simulink model "ElectricVehicleThermalManagementWithHeatPump_2026a_version"  (R2026a)
settings: Solver=VariableStepAuto  StopTime=3600  AbsTol=1e-3
PreLoadFcn:
  | init_nmpc
InitFcn:
  | init_nmpc
model workspace: external: MATLAB File ElectricVehicleThermalManagementWithHeatPumpParameters.m (data not in the file)
values from neighbouring files (symbols this model uses):
  battery_C1_LUT = [1913.6 12447 30609 ... (first row only)    [ElectricVehicleThermalManagementWithHeatPumpParameters.m]
  battery_capacity_LUT = [280.081 276.25 276.392]    [ElectricVehicleThermalManagementWithHeatPumpParameters.m]
  battery_cell_cp = 795    [ElectricVehicleThermalManagementWithHeatPumpParameters.m]
  battery_cell_mass = 2.5    [ElectricVehicleThermalManagementWithHeatPumpParameters.m]
  battery_Em_LUT = [3.4966 3.5057 3.5148 ... (first row only)    [ElectricVehicleThermalManagementWithHeatPumpParameters.m]
  battery_N_cells = 20    [ElectricVehicleThermalManagementWithHeatPumpParameters.m]
  battery_Qe_init = 0    [ElectricVehicleThermalManagementWithHeatPumpParameters.m]
  battery_R0_LUT = [0.0117 0.0085 0.009 ... (first row only)    [ElectricVehicleThermalManagementWithHeatPumpParameters.m]
  battery_R1_LUT = [0.0109 0.0029 0.0013 ... (first row only)    [ElectricVehicleThermalManagementWithHeatPumpParameters.m]
  battery_SOC_LUT = [0; 0.1; 0.25; 0.5; 0.75; 0.9; 1]    [ElectricVehicleThermalManagementWithHeatPumpParameters.m]
  battery_T_init = -5    [ElectricVehicleThermalManagementWithHeatPumpParameters.m]
  battery_temperature_LUT = [5 20 40]    [ElectricVehicleThermalManagementWithHeatPumpParameters.m]
  cabin_duct_area = 0.04    [ElectricVehicleThermalManagementWithHeatPumpParameters.m]
  cabin_T_init = -5    [ElectricVehicleThermalManagementWithHeatPumpParameters.m]
  chiller_area_primary = 0.43982297150257105    (= 0.439822971503)    [ElectricVehicleThermalManagementWithHeatPumpParameters.m]
  chiller_N_baffles = 3    [ElectricVehicleThermalManagementWithHeatPumpParameters.m]
  chiller_N_tubes = 100    [ElectricVehicleThermalManagementWithHeatPumpParameters.m]
  chiller_tube_D = 0.0035    [ElectricVehicleThermalManagementWithHeatPumpParameters.m]
  chiller_tube_L = 0.4    [ElectricVehicleThermalManagementWithHeatPumpParameters.m]
  chiller_wall_conductivity = 240    [ElectricVehicleThermalManagementWithHeatPumpParameters.m]
  chiller_wall_thickness = 0.0001    [ElectricVehicleThermalManagementWithHeatPumpParameters.m]
  cond_evap_air_area_flow = 0.3906    [ElectricVehicleThermalManagementWithHeatPumpParameters.m]
  cond_evap_air_area_primary = 1.4834999999999998    (= 1.4835)    [ElectricVehicleThermalManagementWithHeatPumpParameters.m]
  cond_evap_W = 0.015    [ElectricVehicleThermalManagementWithHeatPumpParameters.m]
  cond_evap_wall_conductivity = 240    [ElectricVehicleThermalManagementWithHeatPumpParameters.m]
  cond_evap_wall_thickness = 0.0001    [ElectricVehicleThermalManagementWithHeatPumpParameters.m]
  coolant_channel_D = 0.0092    [ElectricVehicleThermalManagementWithHeatPumpParameters.m]
  coolant_pipe_D = 0.019    [ElectricVehicleThermalManagementWithHeatPumpParameters.m]
  coolant_T_init = -5    [ElectricVehicleThermalManagementWithHeatPumpParameters.m]
  coolant_tank_area = 0.0121    [ElectricVehicleThermalManagementWithHeatPumpParameters.m]
  coolant_tank_volume = 1.25    [ElectricVehicleThermalManagementWithHeatPumpParameters.m]
  coolant_valve_D_ratio_max = 0.95    [ElectricVehicleThermalManagementWithHeatPumpParameters.m]
  coolant_valve_D_ratio_min = 0.001    [ElectricVehicleThermalManagementWithHeatPumpParameters.m]
  coolant_valve_displacement = 0.0063    [ElectricVehicleThermalManagementWithHeatPumpParameters.m]
  coolant_valve_S_max = 0.0053    [ElectricVehicleThermalManagementWithHeatPumpParameters.m]
  evaporator_air_area_flow = 0.12    [ElectricVehicleThermalManagementWithHeatPumpParameters.m]
  evaporator_air_area_primary = 0.4323    [ElectricVehicleThermalManagementWithHeatPumpParameters.m]
  evaporator_W = 0.015    [ElectricVehicleThermalManagementWithHeatPumpParameters.m]
  evaporator_wall_conductivity = 240    [ElectricVehicleThermalManagementWithHeatPumpParameters.m]
  evaporator_wall_thickness = 0.0001    [ElectricVehicleThermalManagementWithHeatPumpParameters.m]
  expansion_valve_D_ratio_max = 0.9    [ElectricVehicleThermalManagementWithHeatPumpParameters.m]
  hex_area_primary = 0.070371675440411369    (= 0.0703716754404)    [ElectricVehicleThermalManagementWithHeatPumpParameters.m]
  hex_N_tubes = 64    [ElectricVehicleThermalManagementWithHeatPumpParameters.m]
  hex_tube_D = 0.0035    [ElectricVehicleThermalManagementWithHeatPumpParameters.m]
  hex_wall_conductivity = 240    [ElectricVehicleThermalManagementWithHeatPumpParameters.m]
  hex_wall_thickness = 0.0001    [ElectricVehicleThermalManagementWithHeatPumpParameters.m]
  inner_cond_air_area_flow = 0.1953    [ElectricVehicleThermalManagementWithHeatPumpParameters.m]
  inner_cond_air_area_primary = 0.99520000000000008    (= 0.9952)    [ElectricVehicleThermalManagementWithHeatPumpParameters.m]
  inner_cond_W = 0.02    [ElectricVehicleThermalManagementWithHeatPumpParameters.m]
  inner_cond_wall_conductivity = 240    [ElectricVehicleThermalManagementWithHeatPumpParameters.m]
  inner_cond_wall_thickness = 0.0001    [ElectricVehicleThermalManagementWithHeatPumpParameters.m]
  pump_speed_max = 1000    [ElectricVehicleThermalManagementWithHeatPumpParameters.m]
  radiator_air_area_flow = 0.097499999999999989    (= 0.0975)    [ElectricVehicleThermalManagementWithHeatPumpParameters.m]
  radiator_air_area_primary = 0.43687499999999996    (= 0.436875)    [ElectricVehicleThermalManagementWithHeatPumpParameters.m]
  radiator_W = 0.015    [ElectricVehicleThermalManagementWithHeatPumpParameters.m]
  radiator_wall_conductivity = 240    [ElectricVehicleThermalManagementWithHeatPumpParameters.m]
  radiator_wall_thickness = 0.0001    [ElectricVehicleThermalManagementWithHeatPumpParameters.m]
  refrigerant_p_init = 0.25    [ElectricVehicleThermalManagementWithHeatPumpParameters.m]
  refrigerant_pipe_D = 0.01    [ElectricVehicleThermalManagementWithHeatPumpParameters.m]
  refrigerant_valve_D_ratio_max = 0.95    [ElectricVehicleThermalManagementWithHeatPumpParameters.m]
  refrigerant_valve_displacement = 0.005    [ElectricVehicleThermalManagementWithHeatPumpParameters.m]
libraries: fl_lib x227, nesl_utility x162, SimscapeFluids_lib x30, LiBatteryElements_lib x16, slpidlib x3, SignalEditorBlockLib x1
(part 6 of 13)

== system ElectricVehicleThermalManagementWithHeatPump_2026a_version/Inverter ==
  Controlled Heat Flow Rate Source : fl_lib/Thermal/Thermal Sources/Controlled Heat Flow Rate Source
  Coolant Jacket : SimscapeFluids_lib/Thermal Liquid/Pipes & Fittings/Pipe (TL)  dynamic_compressibility=simscape.enum.onoff.on  inertia=simscape.enum.onoff.off  num_segments=1  pipe_length=0.4 m  cross_section_geometry=fluids.thermal_liquid.pipes_fittings.enum.CrossSectionGeometry.Custom  pipe_diameter=0.1 m  pipe_inner_diameter=0.05 m  pipe_outer_diameter=0.1 m  pipe_width=0.1 m  pipe_height=0.1 m  pipe_major_axis=0.1 m  pipe_minor_axis=0.05 m  pipe_side=0.1 m  pipe_angle=30 deg  area=4 * pi * coolant_channel_D^2 / 4 m^2  Dh=coolant_channel_D m  annular_heat_transfer_walls=fluids.thermal_liquid.pipes_fittings.enum.AnnularPipeWalls.AnnularInner  elevation_spec=foundation.enum.constant_variable.constant  elevation_gain=0 m  gravity_spec=foundation.enum.constant_variable.constant  g=9.81 m/s^2  pressure_loss_spec=fluids.thermal_liquid.pipes_fittings.enum.PressureLossSpec.Haaland  local_pressure_loss_spec=fluids.thermal_liquid.pipes_fittings.enum.LocalLossSpec.AggregateLength  length_add=20 * coolant_channel_D * 4 m  loss_coefficient=0.1  roughness_spec=fluids.thermal_liquid.pipes_fittings.enum.RoughnessSpec.Custom  roughness=1.5e-5 m  Re_friction_TLU=[ 400 1000 1.5e+3 3e+3 4e+3 6e+3 1e+4 2e+4 4e+4 6e+4 1e+5 1e+8 ]  friction_factor_TLU=[ 0.264 0.112 0.07099999999999999 0.0417 0.0387 0.0268 0.025 0.0232 0.0226 0.022 0.0214 0.0214 ]  Re_lam=100  Re_tur=500  shape_factor=64  mdot_nominal=[ 0.1 1 ] kg/s  p_diff_nominal=[ 0.001 0.01 ] MPa  mdot_threshold=1e-6 kg/s  wall_spec=fluids.thermal_liquid.pipes_fittings.enum.wall_spec.rigid  vol_expansion_spec=fluids.thermal_liquid.pipes_fittings.enum.VolumeExpansionSpec.Diameter  area_pressure_gain=1e-6 m^2/MPa  static_pressure_TLU=[.1, 1] MPa  area_pressure_gain_TLU=[1e-05, 1.1e-05] m^2  material_behavior_spec=fluids.thermal_liquid.pipes_fittings.enum.PipeMaterialBehavior.Linear  diameter_pressure_gain=1.2e-6 m/MPa  wall_thickness=0.05 m  elastic_modulus=69 GPa  stress_TLU=[276, 310] MPa  strain_TLU=[.004, .02]  stress_assert_action=simscape.enum.assert.action.none  stress_max=400 MPa  poisson_ratio=0.33  wall_time_constant=0.01 s  environment_spec=foundation.enum.pressure_spec.atmospheric  environment_pressure=0.101325 MPa  thermal_expansion=false  alpha_L_wall=24 um/(deltaK*m)  thermal_expansion_Tref=293.15 K  heat_transfer_spec=fluids.thermal_liquid.pipes_fittings.enum.HeatTransferSpec.DittusBoelter  mdot_nominal_heat=[ 0.1 1 ] kg/s  T_in_nominal=[ 293.15 293.15 ] K  T_out_nominal=[ 300 300 ] K  p_in_nominal_heat=[ 0.101325 0.101325 ] MPa  T_wall_nominal=[ 303.15 303.15 ] K  T_wall_eff_nominal=[303.15, 303.15] K  a_coeff=0.3  b_Re_power=0.8  c_Pr_power=0.33  Nu_lam=3.66  Re_Colburn_TLU=[ 100 150 1000 ]  Colburn_factor_TLU=[ 0.019 0.013 0.002 ]  Re_Nu_TLU=[ 100 150 1000 ]  Pr_Nu_TLU=[ 1 10 ]  Nu_TLU=[ 3.72 4.21; 3.75 4.44; 4.21 7.15 ]  annular_correction=fluids.thermal_liquid.pipes_fittings.enum.AnnularPipeCorrectionFactor.Gnielinski  p0_vec=coolant_p_init MPa  T0_vec=coolant_T_init degC  mdot0=0.1 kg/s  p_nominal=0.101325 MPa  T_nominal=293.15 K
  Inverter : fl_lib/Thermal/Thermal Elements/Thermal Mass  mass_type=foundation.enum.constant_variable.constant  mass=1 kg  sp_heat=447 J/kg/K  mass_min=1e-6 kg  num_ports=foundation.enum.numPorts2.one  m_specify=off  m_priority=High  m=1 kg  m_nominal_specify=off  m_nominal_value=1  m_nominal_unit=kg  T_specify=on  T_priority=High  T=coolant_T_init degC  T_nominal_specify=off  T_nominal_value=1  T_nominal_unit=K  Q_specify=off  Q_priority=None  Q=0 W  Q_nominal_specify=off  Q_nominal_value=1  Q_nominal_unit=W
  PS-Simulink Converter : nesl_utility/PS-Simulink Converter  PhysicalDomain=network_engine_domain  SubClassName=ps_output  LeftPortType=input  RightPortType=output  PseudoPeriodic=off  Frequencies=[]  VectorFormat=inherit  Unit=degC  AffineConversion=on
  SC7 : Subsystem
  Scope : Scope
      settings: ActiveDisplayYMinimum=-15.64467  ActiveDisplayYMaximum=40.80204
  Simulink-PS Converter : nesl_utility/Simulink-PS Converter  PhysicalDomain=network_engine_domain  SubClassName=ps_input  LeftPortType=input  RightPortType=output  PseudoPeriodic=off  Frequencies=[]  NoiseDistribution=none  NoiseParameters=[]  Unit=W  AffineConversion=off  FilteringAndDerivatives=provide  SimscapeFilterOrder=1  InputFilterTimeConstant=0.001  UdotUserProvided=0
  Temperature Sensor : fl_lib/Thermal/Thermal Sensors/Temperature Sensor  temperature_measure=foundation.enum.MeasurementReference.absolute
  Thermal Reference : fl_lib/Thermal/Thermal Elements/Thermal Reference
  To Workspace : ToWorkspace  VariableName=Q_inverterMeas  SampleTime=-1
  To Workspace1 : ToWorkspace  VariableName=T_inverterMeas  SampleTime=-1
  A : PMIOPort  Side=Left
  B : PMIOPort  Port=2  Side=Right
  tag scope: T_inverter=global
  wires:
  [Q_inverter] -> To Workspace/1, Simulink-PS Converter/1
  PS-Simulink Converter/1 -> To Workspace1/1, Scope/1, [T_inverter]
  connections:
  Inverter/LConn1 -- Controlled Heat Flow Rate Source/LConn1 -- Temperature Sensor/LConn1 -- Coolant Jacket/LConn2
  SC7/LConn1 -- Coolant Jacket/RConn1
  Controlled Heat Flow Rate Source/RConn2 -- Thermal Reference/LConn1
  SC7/RConn1 -- B/RConn1
  PS-Simulink Converter/LConn1 -- Temperature Sensor/RConn1
  A/RConn1 -- Coolant Jacket/LConn1
  Simulink-PS Converter/RConn1 -- Controlled Heat Flow Rate Source/RConn1

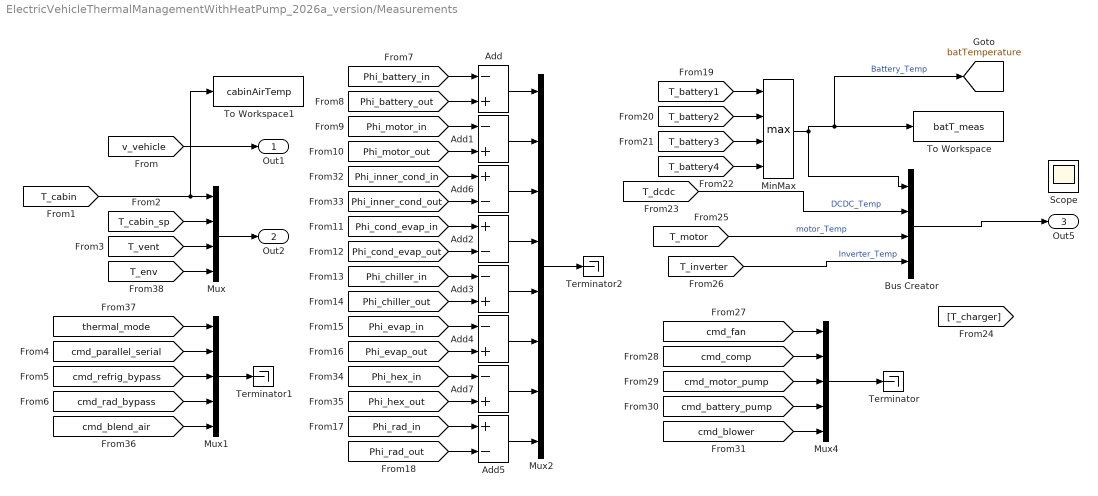
== system ElectricVehicleThermalManagementWithHeatPump_2026a_version/Measurements ==
  Add{,1,3..4,7} (5 alike) : Sum  Inputs=-+
  Add2 : Sum  Inputs=+-
  Add5 : Sum  Inputs=+-
  Add6 : Sum  Inputs=+-
  Bus Creator : BusCreator  Inputs=4
  MinMax : MinMax  Function=max  Inputs=4
  Mux : Mux
  Mux1 : Mux  Inputs=5
  Mux2 : Mux  Inputs=8
  Mux4 : Mux  Inputs=5
  Scope : Scope
      settings: ActiveDisplayYMinimum=-1  ActiveDisplayYMaximum=1  DataLoggingVariableName=ScopeData4
  Terminator : Terminator
  Terminator1 : Terminator
  Terminator2 : Terminator
  To Workspace : ToWorkspace  VariableName=batT_meas  SampleTime=-1
  To Workspace1 : ToWorkspace  VariableName=cabinAirTemp  SampleTime=-1
  Out1 : Outport
  Out2 : Outport  Port=2
  Out5 : Outport  Port=3
  tag scope: batTemperature=global
  wires:
  [v_vehicle] -> Out1/1
  [T_cabin] -> To Workspace1/1, Mux/1
  [T_cabin_sp] -> Mux/2
  [T_vent] -> Mux/3
  Mux/1 -> Out2/1
  Mux1/1 -> Terminator1/1
  [Phi_battery_in] -> Add/1
  [Phi_battery_out] -> Add/2
  [Phi_motor_in] -> Add1/1
  [Phi_motor_out] -> Add1/2
  [Phi_cond_evap_in] -> Add2/1
  [Phi_cond_evap_out] -> Add2/2
  [Phi_chiller_in] -> Add3/1
  [Phi_chiller_out] -> Add3/2
  [Phi_evap_in] -> Add4/1
  [Phi_evap_out] -> Add4/2
  [Phi_rad_in] -> Add5/1
  [Phi_rad_out] -> Add5/2
  Add/1 -> Mux2/1
  Add1/1 -> Mux2/2
  Mux2/1 -> Terminator2/1
  [T_battery1] -> MinMax/1
  [T_battery2] -> MinMax/2
  [T_battery3] -> MinMax/3
  [T_battery4] -> MinMax/4
  [T_dcdc] -> Bus Creator/2  "DCDC_Temp"
  [cmd_fan] -> Mux4/1
  [cmd_comp] -> Mux4/2
  [cmd_motor_pump] -> Mux4/3
  [cmd_battery_pump] -> Mux4/4
  [cmd_blower] -> Mux4/5
  Mux4/1 -> Terminator/1
  [Phi_inner_cond_in] -> Add6/1
  [Phi_inner_cond_out] -> Add6/2
  [Phi_hex_out] -> Add7/2
  [Phi_hex_in] -> Add7/1
  Add5/1 -> Mux2/8
  Add7/1 -> Mux2/7
  Add4/1 -> Mux2/6
  Add3/1 -> Mux2/5
  Add2/1 -> Mux2/4
  Add6/1 -> Mux2/3
  [cmd_blend_air] -> Mux1/5
  [cmd_rad_bypass] -> Mux1/4
  [cmd_refrig_bypass] -> Mux1/3
  [cmd_parallel_serial] -> Mux1/2
  [thermal_mode] -> Mux1/1
  [T_env] -> Mux/4
  MinMax/1 -> Bus Creator/1, [batTemperature], To Workspace/1  "Battery_Temp"
  [T_motor] -> Bus Creator/3  "motor_Temp"
  [T_inverter] -> Bus Creator/4  "Inverter_Temp"
  Bus Creator/1 -> Out5/1

== system ElectricVehicleThermalManagementWithHeatPump_2026a_version/Motor ==
  Controlled Heat Flow Rate Source : fl_lib/Thermal/Thermal Sources/Controlled Heat Flow Rate Source
  Coolant Jacket : SimscapeFluids_lib/Thermal Liquid/Pipes & Fittings/Pipe (TL)  dynamic_compressibility=simscape.enum.onoff.on  inertia=simscape.enum.onoff.off  num_segments=1  pipe_length=0.4 m  cross_section_geometry=fluids.thermal_liquid.pipes_fittings.enum.CrossSectionGeometry.Custom  pipe_diameter=0.1 m  pipe_inner_diameter=0.05 m  pipe_outer_diameter=0.1 m  pipe_width=0.1 m  pipe_height=0.1 m  pipe_major_axis=0.1 m  pipe_minor_axis=0.05 m  pipe_side=0.1 m  pipe_angle=30 deg  area=4 * pi * coolant_channel_D^2 / 4 m^2  Dh=coolant_channel_D m  annular_heat_transfer_walls=fluids.thermal_liquid.pipes_fittings.enum.AnnularPipeWalls.AnnularInner  elevation_spec=foundation.enum.constant_variable.constant  elevation_gain=0 m  gravity_spec=foundation.enum.constant_variable.constant  g=9.81 m/s^2  pressure_loss_spec=fluids.thermal_liquid.pipes_fittings.enum.PressureLossSpec.Haaland  local_pressure_loss_spec=fluids.thermal_liquid.pipes_fittings.enum.LocalLossSpec.AggregateLength  length_add=20 * coolant_channel_D * 4 m  loss_coefficient=0.1  roughness_spec=fluids.thermal_liquid.pipes_fittings.enum.RoughnessSpec.Custom  roughness=1.5e-5 m  Re_friction_TLU=[ 400 1000 1.5e+3 3e+3 4e+3 6e+3 1e+4 2e+4 4e+4 6e+4 1e+5 1e+8 ]  friction_factor_TLU=[ 0.264 0.112 0.07099999999999999 0.0417 0.0387 0.0268 0.025 0.0232 0.0226 0.022 0.0214 0.0214 ]  Re_lam=100  Re_tur=500  shape_factor=64  mdot_nominal=[ 0.1 1 ] kg/s  p_diff_nominal=[ 0.001 0.01 ] MPa  mdot_threshold=1e-6 kg/s  wall_spec=fluids.thermal_liquid.pipes_fittings.enum.wall_spec.rigid  vol_expansion_spec=fluids.thermal_liquid.pipes_fittings.enum.VolumeExpansionSpec.Diameter  area_pressure_gain=1e-6 m^2/MPa  static_pressure_TLU=[.1, 1] MPa  area_pressure_gain_TLU=[1e-05, 1.1e-05] m^2  material_behavior_spec=fluids.thermal_liquid.pipes_fittings.enum.PipeMaterialBehavior.Linear  diameter_pressure_gain=1.2e-6 m/MPa  wall_thickness=0.05 m  elastic_modulus=69 GPa  stress_TLU=[276, 310] MPa  strain_TLU=[.004, .02]  stress_assert_action=simscape.enum.assert.action.none  stress_max=400 MPa  poisson_ratio=0.33  wall_time_constant=0.01 s  environment_spec=foundation.enum.pressure_spec.atmospheric  environment_pressure=0.101325 MPa  thermal_expansion=false  alpha_L_wall=24 um/(deltaK*m)  thermal_expansion_Tref=293.15 K  heat_transfer_spec=fluids.thermal_liquid.pipes_fittings.enum.HeatTransferSpec.DittusBoelter  mdot_nominal_heat=[ 0.1 1 ] kg/s  T_in_nominal=[ 293.15 293.15 ] K  T_out_nominal=[ 300 300 ] K  p_in_nominal_heat=[ 0.101325 0.101325 ] MPa  T_wall_nominal=[ 303.15 303.15 ] K  T_wall_eff_nominal=[303.15, 303.15] K  a_coeff=0.3  b_Re_power=0.8  c_Pr_power=0.33  Nu_lam=3.66  Re_Colburn_TLU=[ 100 150 1000 ]  Colburn_factor_TLU=[ 0.019 0.013 0.002 ]  Re_Nu_TLU=[ 100 150 1000 ]  Pr_Nu_TLU=[ 1 10 ]  Nu_TLU=[ 3.72 4.21; 3.75 4.44; 4.21 7.15 ]  annular_correction=fluids.thermal_liquid.pipes_fittings.enum.AnnularPipeCorrectionFactor.Gnielinski  p0_vec=coolant_p_init MPa  T0_vec=coolant_T_init degC  mdot0=0.1 kg/s  p_nominal=0.101325 MPa  T_nominal=293.15 K
  Motor : fl_lib/Thermal/Thermal Elements/Thermal Mass  mass_type=foundation.enum.constant_variable.constant  mass=46 kg  sp_heat=447 J/kg/K  mass_min=1e-6 kg  num_ports=foundation.enum.numPorts2.one  m_specify=off  m_priority=High  m=1 kg  m_nominal_specify=off  m_nominal_value=1  m_nominal_unit=kg  T_specify=on  T_priority=High  T=coolant_T_init degC  T_nominal_specify=off  T_nominal_value=1  T_nominal_unit=K  Q_specify=off  Q_priority=None  Q=0 W  Q_nominal_specify=off  Q_nominal_value=1  Q_nominal_unit=W
  PS-Simulink Converter : nesl_utility/PS-Simulink Converter  PhysicalDomain=network_engine_domain  SubClassName=ps_output  LeftPortType=input  RightPortType=output  PseudoPeriodic=off  Frequencies=[]  VectorFormat=inherit  Unit=degC  AffineConversion=on
  SC5 : Subsystem
  SC6 : Subsystem
  Simulink-PS Converter : nesl_utility/Simulink-PS Converter  PhysicalDomain=network_engine_domain  SubClassName=ps_input  LeftPortType=input  RightPortType=output  PseudoPeriodic=off  Frequencies=[]  NoiseDistribution=none  NoiseParameters=[]  Unit=W  AffineConversion=off  FilteringAndDerivatives=provide  SimscapeFilterOrder=1  InputFilterTimeConstant=0.001  UdotUserProvided=0
  Temperature Sensor : fl_lib/Thermal/Thermal Sensors/Temperature Sensor  temperature_measure=foundation.enum.MeasurementReference.absolute
  Thermal Reference : fl_lib/Thermal/Thermal Elements/Thermal Reference
  To Workspace : ToWorkspace  VariableName=Q_motMeasured  SampleTime=-1
  To Workspace1 : ToWorkspace  VariableName=Motor_Temp  SampleTime=-1
  A : PMIOPort  Side=Left
  B : PMIOPort  Port=2  Side=Right
  tag scope: T_motor=global
  wires:
  PS-Simulink Converter/1 -> To Workspace1/1, [T_motor]
  [Q_motor] -> To Workspace/1, Simulink-PS Converter/1
  connections:
  Motor/LConn1 -- Coolant Jacket/LConn2 -- Controlled Heat Flow Rate Source/LConn1 -- Temperature Sensor/LConn1
  Simulink-PS Converter/RConn1 -- Controlled Heat Flow Rate Source/RConn1
  PS-Simulink Converter/LConn1 -- Temperature Sensor/RConn1
  SC6/LConn1 -- Coolant Jacket/RConn1
  SC6/RConn1 -- B/RConn1
  SC5/LConn1 -- A/RConn1
  Controlled Heat Flow Rate Source/RConn2 -- Thermal Reference/LConn1
  SC5/RConn1 -- Coolant Jacket/LConn1

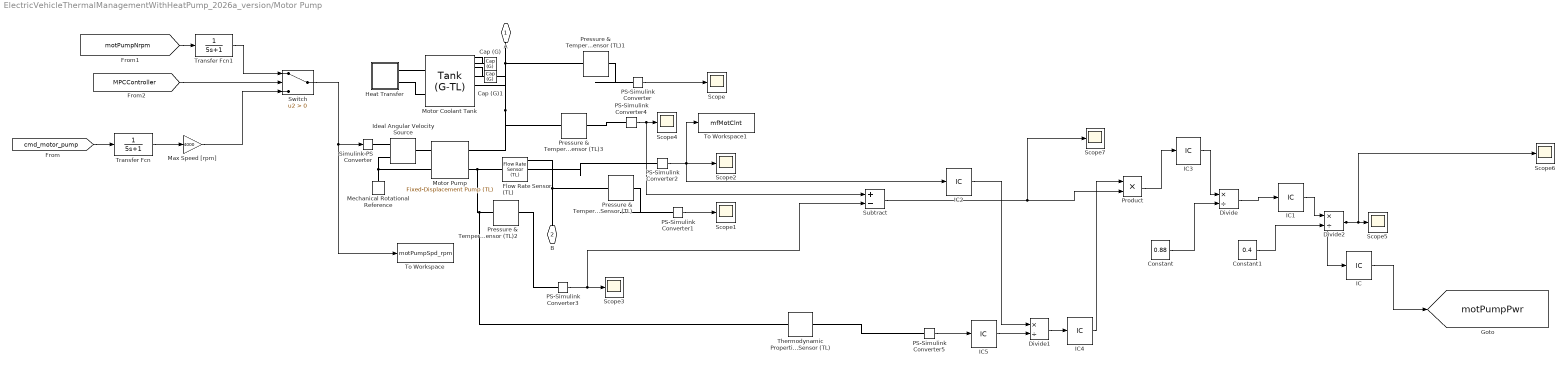
== system ElectricVehicleThermalManagementWithHeatPump_2026a_version/Motor Pump ==
  Cap (G) : fl_lib/Gas/Elements/Cap (G)  p_specify=off  p_priority=None  p=0.101325 MPa  p_nominal_specify=off  p_nominal_value=1  p_nominal_unit=MPa  T_specify=off  T_priority=None  T=293.15 K  T_nominal_specify=off  T_nominal_value=1  T_nominal_unit=K
  Cap (G)1 : fl_lib/Gas/Elements/Cap (G)  p_specify=off  p_priority=None  p=0.101325 MPa  p_nominal_specify=off  p_nominal_value=1  p_nominal_unit=MPa  T_specify=off  T_priority=None  T=293.15 K  T_nominal_specify=off  T_nominal_value=1  T_nominal_unit=K
  Constant : Constant  Value=0.88
  Constant1 : Constant  Value=0.4
  Divide : Product  Inputs=*/
  Divide1 : Product  Inputs=*/
  Divide2 : Product  Inputs=*/
  Flow Rate Sensor (TL) : fl_lib/Thermal Liquid/Sensors/Flow Rate Sensor (TL)  mass_flow_measure=true  volumetric_flow_measure=false  energy_flow_measure=true
  Heat Transfer : Subsystem
  IC{,1..4} (5 alike) : InitialCondition  Value=0
  IC5 : InitialCondition
  Ideal Angular Velocity Source : fl_lib/Mechanical/Mechanical Sources/Ideal Angular Velocity Source
  Max Speed [rpm] : Gain  Gain=4000
  Mechanical Rotational Reference : fl_lib/Mechanical/Rotational Elements/Mechanical Rotational Reference
  Motor Coolant Tank : SimscapeFluids_lib/Thermal Liquid/Tanks & Accumulators/Tank (G-TL)  num_inlet=2  volume_total=coolant_tank_volume l  volume_spec=1  tank_area=coolant_tank_area m^2  level_TLU=[0, 3, 5] m  volume_TLU=[0, 4, 6] m^3  inlet_areas_A1B1=[.01, .01] m^2  inlet_height_A2=0.1 m  inlet_area_A2=0.01 m^2  inlet_heights_A2B2=[0, 0] m  inlet_areas_A2B2=[1 1] * pi * coolant_pipe_D^2 / 4 m^2  inlet_heights_A2B2C2=[.1, .05, 0] m  inlet_areas_A2B2C2=[.01, .01, .01] m^2  inlet_heights_A2B2C2D2=0.1 * ones(1, 4) m  inlet_areas_A2B2C2D2=0.01 * ones(1, 4) m^2  inlet_heights_A2B2C2D2E2=0.1 * ones(1, 5) m  inlet_areas_A2B2C2D2E2=0.01 * ones(1, 5) m^2  inlet_heights_A2B2C2D2E2F2=0.1 * ones(1, 6) m  inlet_areas_A2B2C2D2E2F2=0.01 * ones(1, 6) m^2  capacity_check=0  max_liquid_capacity=coolant_tank_volume l  g=0 m/s^2  level_specify=on  level_priority=None  level=5 m  level_nominal_specify=off  level_nominal_value=1  level_nominal_unit=m  volume_liquid_specify=on  volume_liquid_priority=High  volume_liquid=0.25 * coolant_tank_volume l  volume_liquid_nominal_specify=off  volume_liquid_nominal_value=1  volume_liquid_nominal_unit=m^3  mass_liquid_specify=off  mass_liquid_priority=None  mass_liquid=5e+3 kg  mass_liquid_nominal_specify=off  mass_liquid_nominal_value=1  mass_liquid_nominal_unit=kg  T_liquid_specify=on  T_liquid_priority=High  T_liquid=coolant_T_init degC  T_liquid_nominal_specify=off  T_liquid_nominal_value=1  T_liquid_nominal_unit=K  p_gas_specify=on  p_gas_priority=High  p_gas=coolant_p_init MPa  p_gas_nominal_specify=off  p_gas_nominal_value=1  p_gas_nominal_unit=MPa  T_gas_specify=on  T_gas_priority=High  T_gas=coolant_T_init degC  T_gas_nominal_specify=off  T_gas_nominal_value=1  T_gas_nominal_unit=K  rho_gas_specify=off  rho_gas_priority=None  rho_gas=1.2 kg/m^3  rho_gas_nominal_specify=off  rho_gas_nominal_value=1  rho_gas_nominal_unit=kg/m^3
  Motor Pump : SimscapeFluids_lib/Thermal Liquid/Pumps & Motors/Fixed-Displacement Pump (TL)  loss_spec=1  displacement=pump_displacement l/rev  omega_nominal=0.5 * pump_speed_max rpm  p_nominal=0.1 MPa  mu_nominal=0.9 cP  vol_eff_nominal=0.92  mech_eff_nominal=0.88  no_load_torque=0.03 N*m  p_diff_eff_TLU=[.1, 1, 2] MPa  omega_eff_TLU=[25, 50, 100, 200, 300, 400] rad/s  vol_eff_TLU=[.816, .908, .954, .977, .981, .984; .325, .663, .831, .916, .925, .946; .137, .568, .78, .892, .893, .91]  mech_eff_TLU=[.996, .996, .996, .996, .996, .996; .988, .989, .989, .989, .989, .99; .981, .981, .982, .982, .983, .984]  p_diff_loss_TLU=[.1, 1, 2] MPa  omega_loss_TLU=[25, 50, 100, 200, 300, 400] rad/s  vol_loss_TLU=[.023, .023, .023, .023, .0285, .032; .0844, .0842, .0845, .084, .1125, .108; .1079, .108, .11, .108, .1605, .18] * 1e-3 m^3/s  mech_loss_TLU=[.002, .002, .002, .002, .002, .002; .0607, .0556, .0556, .0556, .0556, .0505; .1937, .1937, .1833, .1833, .1729, .1626] N*m  vol_eff_min=1e-3  vol_eff_max=1  mech_eff_min=1e-3  mech_eff_max=1  pressure_threshold=1e-3 MPa  omega_threshold=10 rad/s  area=pi * coolant_pipe_D^2 / 4 m^2  supplied_range_check=0  pump_mode_check=simscape.enum.assert.action.none  pressure_check=simscape.enum.assert.action.none  p_min_valid=0.101325 MPa
  PS-Simulink Converter{,1..5} (6 alike) : nesl_utility/PS-Simulink Converter  PhysicalDomain=network_engine_domain  SubClassName=ps_output  LeftPortType=input  RightPortType=output  PseudoPeriodic=off  Frequencies=[]  VectorFormat=inherit  Unit=inherit  AffineConversion=off
  Pressure & Temperature Sensor (TL) : fl_lib/Thermal Liquid/Sensors/Pressure & Temperature Sensor (TL)  reference=foundation.enum.MeasurementReference.absolute  pressure=false  pressure_spec=foundation.enum.PressureMeasementSpec.Absolute  temperature=true
  Pressure & Temperature Sensor (TL)1 : fl_lib/Thermal Liquid/Sensors/Pressure & Temperature Sensor (TL)  reference=foundation.enum.MeasurementReference.absolute  pressure=false  pressure_spec=foundation.enum.PressureMeasementSpec.Absolute  temperature=true
  Pressure & Temperature Sensor (TL)2 : fl_lib/Thermal Liquid/Sensors/Pressure & Temperature Sensor (TL)  reference=foundation.enum.MeasurementReference.absolute  pressure=true  pressure_spec=foundation.enum.PressureMeasementSpec.Absolute  temperature=false
  Pressure & Temperature Sensor (TL)3 : fl_lib/Thermal Liquid/Sensors/Pressure & Temperature Sensor (TL)  reference=foundation.enum.MeasurementReference.absolute  pressure=true  pressure_spec=foundation.enum.PressureMeasementSpec.Absolute  temperature=false
  Product : Product
  Scope{,1..7} (8 alike) : Scope
      Scope settings: ActiveDisplayYMinimum=263.0251  ActiveDisplayYMaximum=264.27412  DataLoggingVariableName=ScopeData3
      Scope1 settings: DataLoggingVariableName=ScopeData4
      Scope2 settings: ActiveDisplayYMinimum=-0.01351  ActiveDisplayYMaximum=0.12159  DataLoggingVariableName=ScopeData5
      Scope3 settings: ActiveDisplayYMinimum=100509.25601  ActiveDisplayYMaximum=108666.69589  DataLoggingVariableName=ScopeData3
      Scope4 settings: ActiveDisplayYMinimum=100596.97842  ActiveDisplayYMaximum=107868.3821  DataLoggingVariableName=ScopeData4
      Scope5 settings: ActiveDisplayYMinimum=-0.74504  ActiveDisplayYMaximum=0.24766  DataLoggingVariableName=ScopeData5
      Scope6 settings: DataLoggingVariableName=ScopeData7
      Scope7 settings: ActiveDisplayYMinimum=-0.74504  ActiveDisplayYMaximum=0.24766  DataLoggingVariableName=ScopeData8
  Simulink-PS Converter : nesl_utility/Simulink-PS Converter  PhysicalDomain=network_engine_domain  SubClassName=ps_input  LeftPortType=input  RightPortType=output  PseudoPeriodic=off  Frequencies=[]  NoiseDistribution=none  NoiseParameters=[]  Unit=rpm  AffineConversion=off  FilteringAndDerivatives=provide  SimscapeFilterOrder=1  InputFilterTimeConstant=0.001  UdotUserProvided=0
  Subtract : Sum  Inputs=+-
  Switch : Switch  Criteria=u2 > Threshold  SaturateOnIntegerOverflow=off  InputSameDT=off
  Thermodynamic Properties Sensor (TL) : fl_lib/Thermal Liquid/Sensors/Thermodynamic Properties Sensor (TL)  internal_energy=false  density=true  specific_heat=false
  To Workspace : ToWorkspace  VariableName=motPumpSpd_rpm  SampleTime=-1
  To Workspace1 : ToWorkspace  VariableName=mfMotClnt  SampleTime=-1
  Transfer Fcn : TransferFcn  Denominator=[5 1]
  Transfer Fcn1 : TransferFcn  Denominator=[5 1]
  A : PMIOPort  Side=Left
  B : PMIOPort  Port=2  Side=Right
  tag scope: motPumpPwr=global
  wires:
  Transfer Fcn/1 -> Max Speed [rpm]/1
  [cmd_motor_pump] -> Transfer Fcn/1
  PS-Simulink Converter/1 -> Scope/1
  PS-Simulink Converter1/1 -> Scope1/1
  PS-Simulink Converter2/1 -> IC2/1, To Workspace1/1, Scope2/1
  PS-Simulink Converter3/1 -> Subtract/2, Scope3/1
  PS-Simulink Converter4/1 -> Subtract/1, Scope4/1
  Subtract/1 -> Scope7/1, Product/2
  Product/1 -> IC3/1
  Constant/1 -> Divide/2
  Divide1/1 -> IC4/1
  Constant1/1 -> Divide2/2
  Divide2/1 -> IC/1, Scope6/1, Scope5/1
  PS-Simulink Converter5/1 -> IC5/1
  IC/1 -> [motPumpPwr]
  IC1/1 -> Divide2/1
  Divide/1 -> IC1/1
  IC2/1 -> Divide1/1
  IC3/1 -> Divide/1
  IC4/1 -> Product/1
  IC5/1 -> Divide1/2
  [motPumpNrpm] -> Transfer Fcn1/1
  [MPCController] -> Switch/2
  Max Speed [rpm]/1 -> Switch/3
  Switch/1 -> To Workspace/1, Simulink-PS Converter/1
  Transfer Fcn1/1 -> Switch/1
  connections:
  Mechanical Rotational Reference/LConn1 -- Ideal Angular Velocity Source/RConn2 -- Motor Pump/RConn2
  Ideal Angular Velocity Source/LConn1 -- Motor Pump/RConn1
  Simulink-PS Converter/RConn1 -- Ideal Angular Velocity Source/RConn1
  Pressure & Temperature Sensor (TL)/LConn1 -- Flow Rate Sensor (TL)/RConn1 -- B/RConn1
  Heat Transfer/RConn2 -- Motor Coolant Tank/RConn2
  Cap (G)/LConn1 -- Motor Coolant Tank/LConn1
  Heat Transfer/RConn1 -- Motor Coolant Tank/RConn1
  Motor Coolant Tank/LConn4 -- Pressure & Temperature Sensor (TL)3/LConn1 -- Motor Pump/LConn1
  A/RConn1 -- Pressure & Temperature Sensor (TL)1/LConn1 -- Motor Coolant Tank/LConn3
  Cap (G)1/LConn1 -- Motor Coolant Tank/LConn2
  PS-Simulink Converter/LConn1 -- Pressure & Temperature Sensor (TL)1/RConn1
  PS-Simulink Converter1/LConn1 -- Pressure & Temperature Sensor (TL)/RConn1
  Flow Rate Sensor (TL)/LConn1 -- Thermodynamic Properties Sensor (TL)/LConn1 -- Pressure & Temperature Sensor (TL)2/LConn1 -- Motor Pump/LConn2
  PS-Simulink Converter2/LConn1 -- Flow Rate Sensor (TL)/RConn2
  PS-Simulink Converter3/LConn1 -- Pressure & Temperature Sensor (TL)2/RConn1
  Pressure & Temperature Sensor (TL)3/RConn1 -- PS-Simulink Converter4/LConn1
  PS-Simulink Converter5/LConn1 -- Thermodynamic Properties Sensor (TL)/RConn1

== system ElectricVehicleThermalManagementWithHeatPump_2026a_version/Parallel-Serial Mode Valve 1 ==
  note: Parallel mode flow path: A-C
      | Serial mode flow path: A-B
  Bias : Bias  Bias=-1  SaturateOnIntegerOverflow=off
  Gain : Gain  Gain=2
  Max Valve Displacement [m] : Gain  Gain=coolant_valve_displacement
  Parallel-Serial Mode Valve : SimscapeFluids_lib/Thermal Liquid/Valves & Orifices/Directional Control Valves/3-Way Directional Valve (TL)  open_orifices_pos=fluids.thermal_liquid.valves.directional_control_valves.enum.OpenOrifices3Way.PA  open_orifices_neg=fluids.thermal_liquid.valves.directional_control_valves.enum.OpenOrifices3Way.AT  area_spec=fluids.thermal_liquid.valves.directional_control_valves.enum.area_spec.identical  valve_spec=fluids.thermal_liquid.valves.enum.orifice_spec.linear  del_S_max=coolant_valve_displacement m  area_max=pi * (coolant_valve_D_ratio_max*coolant_pipe_D)^2 / 4 m^2  del_S_TLU=[0 0.002 0.004 0.007 0.017] m  valve_area_TLU=[1e-09, 2.0352e-07, 4.0736e-05, .00011438, .00034356] m^2  del_S_flow_TLU=[0 0.002 0.004 0.007 0.017] m  p_diff_TLU=[-.1, .3, .5, .7] MPa  vol_flow_TLU=1e-3 * [1.7e-05, 2e-05, 2.6e-05; .0035, .0045, .0053; .7, .9, 1.06; 1.96, 2.5, 3; 6, 7.7, 9.13] m^3/s  mdot_TLU=[-1e-05, 1.7e-05, 2e-05, 2.6e-05; -.002, .0035, .0045, .0053; -.4, .7, .9, 1.06; -1.13, 1.96, 2.5, 3; -3.45, 6, 7.7, 9.13] kg/s  T_ref_in=293.15 K  p_ref_in=0.101325 MPa  area_leak=pi * (coolant_valve_D_ratio_min*coolant_pipe_D)^2 / 4 m^2  Cd=0.7  Re_c=150  smoothing_factor=0.01  pressure_recovery=simscape.enum.onoff.on  area=pi * coolant_pipe_D^2 / 4 m^2  S_max_PA=coolant_valve_S_max m  del_S_max_PA=coolant_valve_displacement-(coolant_valve_displacement)*(pi * (coolant_valve_D_ratio_min*coolant_pipe_D)^2 / 4)/(pi * (coolant_valve_D_ratio_max*coolant_pipe_D)^2 / 4) m  area_max_PA=pi * (coolant_valve_D_ratio_max*coolant_pipe_D)^2 / 4 m^2  del_S_TLU_PA=[0 0.002 0.004 0.007 0.017] m  valve_area_TLU_PA=[1e-09, 2.0352e-07, 4.0736e-05, .00011438, .00034356] m^2  del_S_flow_TLU_PA=[0 0.002 0.004 0.007 0.017] m  p_diff_TLU_PA=[-.1, .3, .5, .7] MPa  vol_flow_TLU_PA=1e-3 * [1.7e-05, 2e-05, 2.6e-05; .0035, .0045, .0053; .7, .9, 1.06; 1.96, 2.5, 3; 6, 7.7, 9.13] m^3/s  mdot_TLU_PA=[-1e-05, 1.7e-05, 2e-05, 2.6e-05; -.002, .0035, .0045, .0053; -.4, .7, .9, 1.06; -1.13, 1.96, 2.5, 3; -3.45, 6, 7.7, 9.13] kg/s  S_max_AT=-coolant_valve_S_max m  del_S_max_AT=coolant_valve_displacement-(coolant_valve_displacement)*(pi * (coolant_valve_D_ratio_min*coolant_pipe_D)^2 / 4)/(pi * (coolant_valve_D_ratio_max*coolant_pipe_D)^2 / 4) m  area_max_AT=pi * (coolant_valve_D_ratio_max*coolant_pipe_D)^2 / 4 m^2  del_S_TLU_AT=[0 0.002 0.004 0.007 0.017] m  valve_area_TLU_AT=[1e-09, 2.0352e-07, 4.0736e-05, .00011438, .00034356] m^2  del_S_flow_TLU_AT=[0 0.002 0.004 0.007 0.017] m  p_diff_TLU_AT=[-.1, .3, .5, .7] MPa  vol_flow_TLU_AT=1e-3 * [1.7e-05, 2e-05, 2.6e-05; .0035, .0045, .0053; .7, .9, 1.06; 1.96, 2.5, 3; 6, 7.7, 9.13] m^3/s  mdot_TLU_AT=[-1e-05, 1.7e-05, 2e-05, 2.6e-05; -.002, .0035, .0045, .0053; -.4, .7, .9, 1.06; -1.13, 1.96, 2.5, 3; -3.45, 6, 7.7, 9.13] kg/s  S_max_PT=2.5e-3 m  del_S_max_PT=0.005 m  area_max_PT=1e-4 m^2  del_S_TLU_PT=[0, .002, .004, .007, .017] m  valve_area_TLU_PT=[1e-09, 2.0352e-07, 4.0736e-05, .00011438, .00034356] m^2  del_S_flow_TLU_PT=[0, .002, .004, .007, .017] m  p_diff_TLU_PT=[.3, .5, .7] MPa  vol_flow_TLU_PT=1e-3 * [1.7e-05, 2e-05, 2.6e-05; .0035, .0045, .0053; .7, .9, 1.06; 1.96, 2.5, 3; 6, 7.7, 9.13] m^3/s  mdot_TLU_PT=[1.7e-05, 2e-05, 2.6e-05; .0035, .0045, .0053; .7, .9, 1.06; 1.96, 2.5, 3; 6, 7.7, 9.13] kg/s
  Simulink-PS Converter : nesl_utility/Simulink-PS Converter  PhysicalDomain=network_engine_domain  SubClassName=ps_input  LeftPortType=input  RightPortType=output  PseudoPeriodic=off  Frequencies=[]  NoiseDistribution=none  NoiseParameters=[]  Unit=m  AffineConversion=off  FilteringAndDerivatives=provide  SimscapeFilterOrder=1  InputFilterTimeConstant=0.001  UdotUserProvided=0
  Transfer Fcn : TransferFcn  Denominator=[1 1]
  C : PMIOPort  Side=Left
  A : PMIOPort  Port=2  Side=Right
  B : PMIOPort  Port=3  Side=Right
  wires:
  Gain/1 -> Bias/1
  Transfer Fcn/1 -> Gain/1
  [cmd_parallel_serial] -> Transfer Fcn/1
  Max Valve Displacement [m]/1 -> Simulink-PS Converter/1
  Bias/1 -> Max Valve Displacement [m]/1
  connections:
  Parallel-Serial Mode Valve/RConn1 -- Simulink-PS Converter/RConn1
  Parallel-Serial Mode Valve/RConn3 -- C/RConn1
  Parallel-Serial Mode Valve/LConn1 -- A/RConn1
  Parallel-Serial Mode Valve/RConn2 -- B/RConn1

== system ElectricVehicleThermalManagementWithHeatPump_2026a_version/Parallel-Serial Mode Valve 2 ==
  note: Parallel mode flow path: A-C
      | Serial mode flow path: A-B
  Bias : Bias  Bias=-1  SaturateOnIntegerOverflow=off
  Flow Rate Sensor (TL) : fl_lib/Thermal Liquid/Sensors/Flow Rate Sensor (TL)  mass_flow_measure=true  volumetric_flow_measure=false  energy_flow_measure=true
  Gain : Gain  Gain=2
  Max Valve Displacement [m] : Gain  Gain=coolant_valve_displacement
  PS-Simulink Converter : nesl_utility/PS-Simulink Converter  PhysicalDomain=network_engine_domain  SubClassName=ps_output  LeftPortType=input  RightPortType=output  PseudoPeriodic=off  Frequencies=[]  VectorFormat=inherit  Unit=inherit  AffineConversion=off
  Parallel-Serial Mode Valve : SimscapeFluids_lib/Thermal Liquid/Valves & Orifices/Directional Control Valves/3-Way Directional Valve (TL)  open_orifices_pos=fluids.thermal_liquid.valves.directional_control_valves.enum.OpenOrifices3Way.PA  open_orifices_neg=fluids.thermal_liquid.valves.directional_control_valves.enum.OpenOrifices3Way.AT  area_spec=fluids.thermal_liquid.valves.directional_control_valves.enum.area_spec.identical  valve_spec=fluids.thermal_liquid.valves.enum.orifice_spec.linear  del_S_max=coolant_valve_displacement m  area_max=pi * (coolant_valve_D_ratio_max*coolant_pipe_D)^2 / 4 m^2  del_S_TLU=[0 0.002 0.004 0.007 0.017] m  valve_area_TLU=[1e-09, 2.0352e-07, 4.0736e-05, .00011438, .00034356] m^2  del_S_flow_TLU=[0 0.002 0.004 0.007 0.017] m  p_diff_TLU=[-.1, .3, .5, .7] MPa  vol_flow_TLU=1e-3 * [1.7e-05, 2e-05, 2.6e-05; .0035, .0045, .0053; .7, .9, 1.06; 1.96, 2.5, 3; 6, 7.7, 9.13] m^3/s  mdot_TLU=[-1e-05, 1.7e-05, 2e-05, 2.6e-05; -.002, .0035, .0045, .0053; -.4, .7, .9, 1.06; -1.13, 1.96, 2.5, 3; -3.45, 6, 7.7, 9.13] kg/s  T_ref_in=293.15 K  p_ref_in=0.101325 MPa  area_leak=pi * (coolant_valve_D_ratio_min*coolant_pipe_D)^2 / 4 m^2  Cd=0.7  Re_c=150  smoothing_factor=0.01  pressure_recovery=simscape.enum.onoff.on  area=pi * coolant_pipe_D^2 / 4 m^2  S_max_PA=coolant_valve_S_max m  del_S_max_PA=coolant_valve_displacement-(coolant_valve_displacement)*(pi * (coolant_valve_D_ratio_min*coolant_pipe_D)^2 / 4)/(pi * (coolant_valve_D_ratio_max*coolant_pipe_D)^2 / 4) m  area_max_PA=pi * (coolant_valve_D_ratio_max*coolant_pipe_D)^2 / 4 m^2  del_S_TLU_PA=[0 0.002 0.004 0.007 0.017] m  valve_area_TLU_PA=[1e-09, 2.0352e-07, 4.0736e-05, .00011438, .00034356] m^2  del_S_flow_TLU_PA=[0 0.002 0.004 0.007 0.017] m  p_diff_TLU_PA=[-.1, .3, .5, .7] MPa  vol_flow_TLU_PA=1e-3 * [1.7e-05, 2e-05, 2.6e-05; .0035, .0045, .0053; .7, .9, 1.06; 1.96, 2.5, 3; 6, 7.7, 9.13] m^3/s  mdot_TLU_PA=[-1e-05, 1.7e-05, 2e-05, 2.6e-05; -.002, .0035, .0045, .0053; -.4, .7, .9, 1.06; -1.13, 1.96, 2.5, 3; -3.45, 6, 7.7, 9.13] kg/s  S_max_AT=-coolant_valve_S_max m  del_S_max_AT=coolant_valve_displacement-(coolant_valve_displacement)*(pi * (coolant_valve_D_ratio_min*coolant_pipe_D)^2 / 4)/(pi * (coolant_valve_D_ratio_max*coolant_pipe_D)^2 / 4) m  area_max_AT=pi * (coolant_valve_D_ratio_max*coolant_pipe_D)^2 / 4 m^2  del_S_TLU_AT=[0 0.002 0.004 0.007 0.017] m  valve_area_TLU_AT=[1e-09, 2.0352e-07, 4.0736e-05, .00011438, .00034356] m^2  del_S_flow_TLU_AT=[0 0.002 0.004 0.007 0.017] m  p_diff_TLU_AT=[-.1, .3, .5, .7] MPa  vol_flow_TLU_AT=1e-3 * [1.7e-05, 2e-05, 2.6e-05; .0035, .0045, .0053; .7, .9, 1.06; 1.96, 2.5, 3; 6, 7.7, 9.13] m^3/s  mdot_TLU_AT=[-1e-05, 1.7e-05, 2e-05, 2.6e-05; -.002, .0035, .0045, .0053; -.4, .7, .9, 1.06; -1.13, 1.96, 2.5, 3; -3.45, 6, 7.7, 9.13] kg/s  S_max_PT=2.5e-3 m  del_S_max_PT=0.005 m  area_max_PT=1e-4 m^2  del_S_TLU_PT=[0, .002, .004, .007, .017] m  valve_area_TLU_PT=[1e-09, 2.0352e-07, 4.0736e-05, .00011438, .00034356] m^2  del_S_flow_TLU_PT=[0, .002, .004, .007, .017] m  p_diff_TLU_PT=[.3, .5, .7] MPa  vol_flow_TLU_PT=1e-3 * [1.7e-05, 2e-05, 2.6e-05; .0035, .0045, .0053; .7, .9, 1.06; 1.96, 2.5, 3; 6, 7.7, 9.13] m^3/s  mdot_TLU_PT=[1.7e-05, 2e-05, 2.6e-05; .0035, .0045, .0053; .7, .9, 1.06; 1.96, 2.5, 3; 6, 7.7, 9.13] kg/s
  Scope : Scope
      settings: ActiveDisplayYMinimum=-1  ActiveDisplayYMaximum=1  DataLoggingVariableName=ScopeData3
  Simulink-PS Converter : nesl_utility/Simulink-PS Converter  PhysicalDomain=network_engine_domain  SubClassName=ps_input  LeftPortType=input  RightPortType=output  PseudoPeriodic=off  Frequencies=[]  NoiseDistribution=none  NoiseParameters=[]  Unit=m  AffineConversion=off  FilteringAndDerivatives=provide  SimscapeFilterOrder=1  InputFilterTimeConstant=0.001  UdotUserProvided=0
  Transfer Fcn : TransferFcn  Denominator=[1 1]
  A : PMIOPort  Side=Left
  B : PMIOPort  Port=2  Side=Left
  C : PMIOPort  Port=3  Side=Right
  wires:
  Bias/1 -> Max Valve Displacement [m]/1
  [cmd_parallel_serial] -> Transfer Fcn/1
  Gain/1 -> Bias/1
  Max Valve Displacement [m]/1 -> Simulink-PS Converter/1
  Transfer Fcn/1 -> Gain/1
  PS-Simulink Converter/1 -> Scope/1
  connections:
  Parallel-Serial Mode Valve/RConn3 -- C/RConn1
  Parallel-Serial Mode Valve/LConn1 -- Flow Rate Sensor (TL)/LConn1 -- A/RConn1
  Parallel-Serial Mode Valve/RConn2 -- B/RConn1
  Simulink-PS Converter/RConn1 -- Parallel-Serial Mode Valve/RConn1
  PS-Simulink Converter/LConn1 -- Flow Rate Sensor (TL)/RConn2
